simulink model "IMU_Filter"  (R2026a)
settings: Solver=VariableStepAuto
undefined symbols (not defined in the file or in its folder): LF
libraries: simulink x3, instrumentseriallib x2
settings Model: Creator=jamie  LastModifiedBy=root

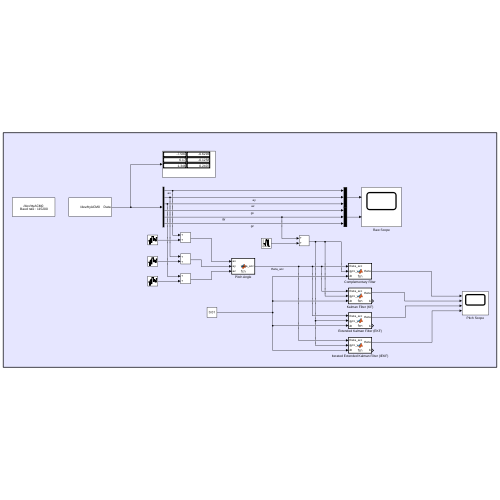
[thumbnail: Simulink's stored preview of the top-level diagram]
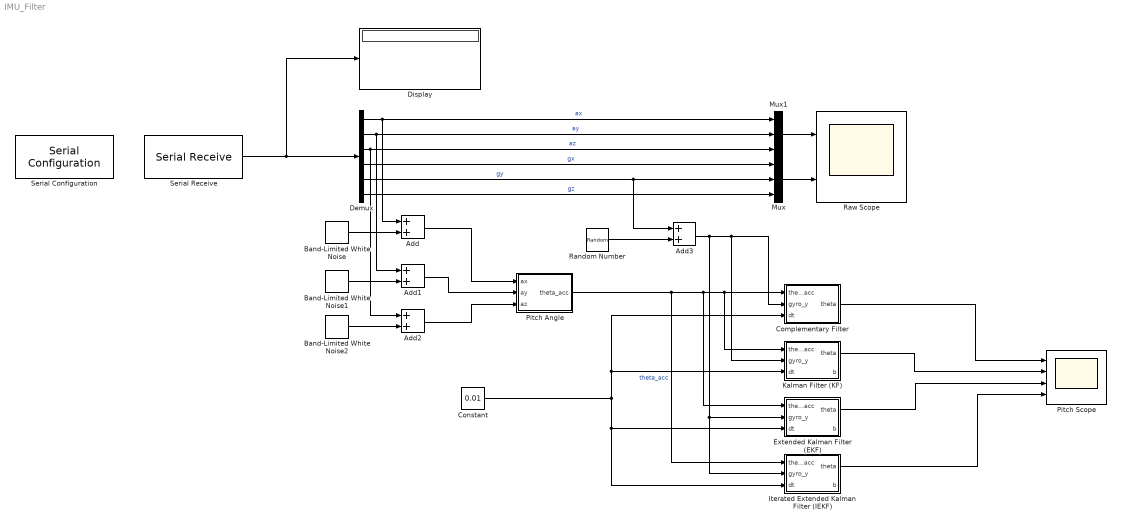
== system IMU_Filter ==
  Add{,1..3} (4 alike) : Sum
  Band-Limited White Noise : simulink/Sources/Band-Limited White Noise  Cov=[0.1]  Ts=0.01  seed=[23341]
  Band-Limited White Noise1 : simulink/Sources/Band-Limited White Noise  Cov=[0.1]  Ts=0.01  seed=[24341]
  Band-Limited White Noise2 : simulink/Sources/Band-Limited White Noise  Cov=[0.1]  Ts=0.01  seed=[24741]
  Complementary Filter : MATLAB Function  TreatAsAtomicUnit=on
  Constant : Constant  Value=0.01
  Demux : Demux  Outputs=6
  Display : Display
  Extended Kalman Filter (EKF) : MATLAB Function  TreatAsAtomicUnit=on
  Iterated Extended Kalman Filter (IEKF) : MATLAB Function  TreatAsAtomicUnit=on
  Kalman Filter (KF) : MATLAB Function  TreatAsAtomicUnit=on
  Mux : Mux  Inputs=3
  Mux1 : Mux  Inputs=3
  Pitch Angle : MATLAB Function  TreatAsAtomicUnit=on
  Pitch Scope : Scope  NumInputPorts=4
      settings: ActiveDisplayYMinimum=-12.645169837667602  ActiveDisplayYMaximum=6.1412368347517088
  Random Number : RandomNumber  Mean=0.005  Variance=0.001  Seed=1324  SampleTime=0.01
  Raw Scope : Scope  NumInputPorts=2
      settings: ActiveDisplayYMinimum=-9.4165056943893433  ActiveDisplayYMaximum=14.411522746086121
  Serial Configuration : instrumentseriallib/Serial Configuration  Priority=-200000  PortSel=/dev/ttyACM0  Port=/dev/ttyACM0  ComPort=/dev/ttyACM0  BaudRate=115200  DataBits=8  Parity=none  StopBits=1  ByteOrder=little-endian  FlowControl=none  Timeout=10  SimulateUsing=Interpreted execution  BlockInModel=on  aMode=1
  Serial Receive : instrumentseriallib/Serial Receive  Priority=1  PortSel=/dev/ttyACM0  Port=/dev/ttyACM0  ComPort=/dev/ttyACM0  DataType=single  SaveDataType=uint8  ToggleHeader=off  Header=[]  ToggleDataSize=on  DataSize=[1, 6]  ToggleTerminator=off  Terminator=LF ('\n')  CustomTerminator=[]  InputFormat=Column major  EnableBlockingMode=on  ActionDataUnavailable=Output last received value  ActionWhenDataUnavailable=Output last received value  CustomValue=0  SampleTime=0.01  SimulateUsing=Interpreted execution  BlockInModel=on  aMode=1  LibraryInUse=instrumentlib
  wires:
  Serial Receive/1 -> Demux/1, Display/1
  Demux/4 -> Mux/1  "gx"
  Demux/6 -> Mux/3  "gz"
  Demux/3 -> Add2/1, Mux1/3  "az"
  Demux/1 -> Mux1/1, Add/1  "ax"
  Demux/2 -> Add1/1, Mux1/2  "ay"
  Mux/1 -> Raw Scope/2
  Mux1/1 -> Raw Scope/1
  Pitch Angle/1(theta_acc) -> Extended Kalman Filter (EKF)/1(theta_acc), Kalman Filter (KF)/1(theta_acc), Complementary Filter/1(theta_acc), Iterated Extended Kalman Filter (IEKF)/1(theta_acc)  "theta_acc"
  Complementary Filter/1(theta) -> Pitch Scope/1
  Kalman Filter (KF)/1(theta) -> Pitch Scope/2
  Extended Kalman Filter (EKF)/1(theta) -> Pitch Scope/3
  Iterated Extended Kalman Filter (IEKF)/1(theta) -> Pitch Scope/4
  Constant/1 -> Iterated Extended Kalman Filter (IEKF)/3(dt), Extended Kalman Filter (EKF)/3(dt), Kalman Filter (KF)/3(dt), Complementary Filter/3(dt)
  Band-Limited White Noise/1 -> Add/2
  Add/1 -> Pitch Angle/1(ax)
  Band-Limited White Noise2/1 -> Add2/2
  Band-Limited White Noise1/1 -> Add1/2
  Add1/1 -> Pitch Angle/2(ay)
  Add2/1 -> Pitch Angle/3(az)
  Demux/5 -> Add3/1, Mux/2  "gy"
  Random Number/1 -> Add3/2
  Add3/1 -> Iterated Extended Kalman Filter (IEKF)/2(gyro_y), Extended Kalman Filter (EKF)/2(gyro_y), Kalman Filter (KF)/2(gyro_y), Complementary Filter/2(gyro_y)

== matlab function IMU_Filter/Complementary Filter ==
  data: theta_acc input; theta output; gyro_y input; dt input
function theta = fcn(theta_acc, gyro_y, dt)
    theta_acc = double(theta_acc);
    gyro_y    = double(gyro_y);
    dt        = double(dt);

    % Set up the previous theta value
    persistent theta_prev
    if isempty(theta_prev)
        theta_prev = 0;
    end
    
    % Complementary filter w/ high-pass gyro + low-pass accelerometer
    alpha = 0.98;
    theta = alpha * (theta_prev + gyro_y * dt) + (1 - alpha) * theta_acc;
    theta_prev = theta;
end

== matlab function IMU_Filter/Pitch Angle ==
  data: ax input; theta_acc output; ay input; az input
function theta_acc = fcn(ax, ay, az)
    % Calculate pitch angle in radians from static acceleration
    theta_acc = atan2(ax, sqrt(ay^2 + az^2));
end

== matlab function IMU_Filter/Kalman Filter (KF) ==
  data: theta_acc input; theta output; gyro_y input; dt input; b output
function [theta, b] = fcn(theta_acc, gyro_y, dt)
    theta_acc = double(theta_acc);
    gyro_y    = double(gyro_y);
    dt        = double(dt);

    persistent x P
    if isempty(x)
        x = [0; 0];
        P = eye(2);
    end

    % --- EMPIRICAL COVARIANCE MATRICES ---
    R = 0.00000382;
    Q = [4.0e-10 , 0 ;
         0       , 1.0e-6];
    % ------------------------------------

    A = [1, -dt; 0, 1];
    B = [dt; 0];
    C = [1, 0];
    
    % Predict
    x_pred = A * x + B * gyro_y;
    P_pred = A * P * A' + Q;
    
    % Update
    K = (P_pred * C') / (C * P_pred * C' + R);
    x = x_pred + K * (theta_acc - C * x_pred);
    P = (eye(2) - K * C) * P_pred;
    
    % Clamp the angle back to [-pi, pi] interval after the state update
    x(1) = atan2(sin(x(1)), cos(x(1)));

    theta = x(1);
    b     = x(2);
end

== matlab function IMU_Filter/Iterated Extended Kalman Filter (IEKF) ==
  data: theta_acc input; theta output; gyro_y input; dt input; b output
function [theta, b] = fcn(theta_acc, gyro_y, dt)
    theta_acc = double(theta_acc);
    gyro_y    = double(gyro_y);
    dt        = double(dt);

    persistent x P
    if isempty(x)
        x = [0; 0];
        P = eye(2);
    end

    % --- EMPIRICAL COVARIANCE MATRICES ---
    R = 0.00000382;
    Q = [4.0e-10 , 0 ;
         0       , 1.0e-6];
    % ------------------------------------

    A = [1, -dt; 0, 1];
    B = [dt; 0];
    
    % Predict
    x_pred = A * x + B * gyro_y;
    P_pred = A * P * A' + Q;
    
    % Iterated Update Loop
    eta = x_pred;
    num_iters = 4;
    for i = 1:num_iters
        H = [cos(eta(1)), 0];
        h_eta = sin(eta(1));
        
        K = (P_pred * H') / (H * P_pred * H' + R);
        eta = x_pred + K * (sin(theta_acc) - h_eta - H * (x_pred - eta));
    end
    
    x = eta;
    P = (eye(2) - K * H) * P_pred;
    
    % Clamp the angle back to [-pi, pi] interval after the state update
    x(1) = atan2(sin(x(1)), cos(x(1)));

    theta = x(1);
    b     = x(2);
end

== matlab function IMU_Filter/Extended Kalman Filter (EKF) ==
  data: theta_acc input; theta output; gyro_y input; dt input; b output
function [theta, b] = fcn(theta_acc, gyro_y, dt)
    theta_acc = double(theta_acc);
    gyro_y    = double(gyro_y);
    dt        = double(dt);

    persistent x P
    if isempty(x)
        x = [0; 0];
        P = eye(2);
    end

    % --- EMPIRICAL COVARIANCE MATRICES ---
    R = 0.00000382;
    Q = [4.0e-10 , 0 ;
         0       , 1.0e-6];
    % ------------------------------------

    A = [1, -dt; 0, 1];
    B = [dt; 0];
    
    % Predict
    x_pred = A * x + B * gyro_y;
    P_pred = A * P * A' + Q;
    
    % Non-linear Update (Single Pass)
    H = [cos(x_pred(1)), 0];
    y_tilde = sin(theta_acc) - sin(x_pred(1));
    
    K = (P_pred * H') / (H * P_pred * H' + R);
    x = x_pred + K * y_tilde;
    P = (eye(2) - K * H) * P_pred;
    
    % Clamp the angle back to [-pi, pi] interval after the state update
    x(1) = atan2(sin(x(1)), cos(x(1)));

    theta = x(1);
    b     = x(2);
end
